simulink model "HIamp_record_LSL_DD_vMMR"  (R2020a)
settings: Solver=FixedStepDiscrete  StartTime=0.0  StopTime=10000  FixedStep=1/600  RelTol=1e-3
InitFcn:
  | % Added for LSL timestamp logging (see README, "LSL timestamps").
  | % 1) put the model folder on the path so LSLMarkerTimestamps.m is found;
  | % 2) name the timing file after the EEG file: <EEG name>_LSLtiming.mat
  | addpath(fileparts(get_param(bdroot, 'FileName')));
  | [p_, n_, e_] = fileparts(get_param([bdroot '/To File'], 'Filename'));
  | set_param([bdroot '/To File LSL timing'], 'Filename', fullfile(p_, [n_ '_LSLtiming' e_]));
  | fprintf('LSL timing file: %s\n', get_param([bdroot '/To File LSL timing'], 'Filename'));
  | clear p_ n_ e_
libraries: LSL x1, DataAcquisition x1
settings Model: Creator=AvivaLab  LastModifiedBy=AvivaLab
settings SolverCC: AutoInsertRateTranBlk=on

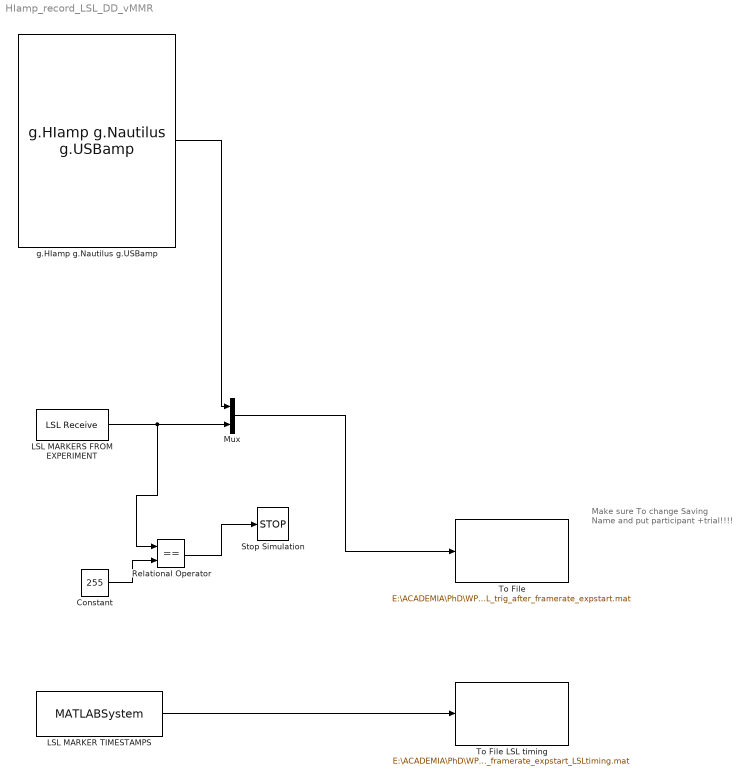
== system HIamp_record_LSL_DD_vMMR ==
  note: Make sure To change Saving Name and put participant +trial!!!!
  Constant : Constant  Value=255
  LSL MARKER TIMESTAMPS : MATLABSystem  System=LSLMarkerTimestamps  StreamName=experiment_markers  ResolveTimeout=5  CorrectionInterval=1  SimulateUsing=Interpreted execution
      mask Type: LSLMarkerTimestamps
      mask Display:
      | disp('LSLMarkerTimestamps');
      | port_label('output',1,'y');
  LSL MARKERS FROM EXPERIMENT : LSL/LSL Receive  noChannels=1  lslPropName=name  lslPropValue='experiment_markers'  sampleRate=600
      settings: SourceProductName=g.HIsys
  Mux : Mux  Inputs=2
  Relational Operator : RelationalOperator  Operator===  OutDataTypeStr=boolean  RndMeth=Simplest
  Stop Simulation : Stop
  To File : ToFile  Filename=E:\ACADEMIA\PhD\WP5\EEG_Recordings\Photodiode_Calib_vMMR\photodiode_test_20261013_8_slx_frame_length_4_timestamped_LSL_trig_after_framerate_expstart.mat  MatrixName=EEG_data
  To File LSL timing : ToFile  Filename=E:\ACADEMIA\PhD\WP5\EEG_Recordings\Photodiode_Calib_vMMR\photodiode_test_20261013_8_slx_frame_length_4_timestamped_LSL_trig_after_framerate_expstart_LSLtiming.mat  MatrixName=LSL_timing  SaveFormat=Timeseries
  g.HIamp g.Nautilus g.USBamp : DataAcquisition/g.HIamp g.Nautilus g.USBamp  cfgUpdated=740268.506  numDevices=2  deviceSR=[500 250 ]  deviceChannels=[9 4 ]  numSR=[2 ]  SRIndexPerDevice=[1 0 ]
      settings: SourceProductName=g.HIsys
  wires:
  g.HIamp g.Nautilus g.USBamp/1 -> Mux/1
  LSL MARKERS FROM EXPERIMENT/1 -> Relational Operator/1, Mux/2
  Mux/1 -> To File/1
  Relational Operator/1 -> Stop Simulation/1
  Constant/1 -> Relational Operator/2
  LSL MARKER TIMESTAMPS/1 -> To File LSL timing/1
